simulink model "Hopper_3DOF_v1_9_J"  (R2025a)
settings: Solver=VariableStepAuto  StartTime=0.0  StopTime=20  RelTol=1e-3
values from neighbouring files (symbols this model uses):
  g = 9.80665    [vehicle_info.m]
  I = [ I_xx, 0,     0 ... (first row only)    [vehicle_info.m]
  m0 = 48    [vehicle_info.m]
  mdot = 0    [vehicle_info.m]
  mt = 114    [vehicle_info.m]
undefined symbols (not defined in the file or in its folder): bp, tbl
libraries: aerolibanim x3, aerolibobsolete x1, simulink_extras x1, slpidlib x1, simulink x1, SignalEditorBlockLib x1
settings Model: Creator=vip  LastModifiedBy=asing
settings SolverCC: ZeroCrossAlgorithm=Adaptive
settings DebuggingCC: IgnoredZcDiagnostic=none

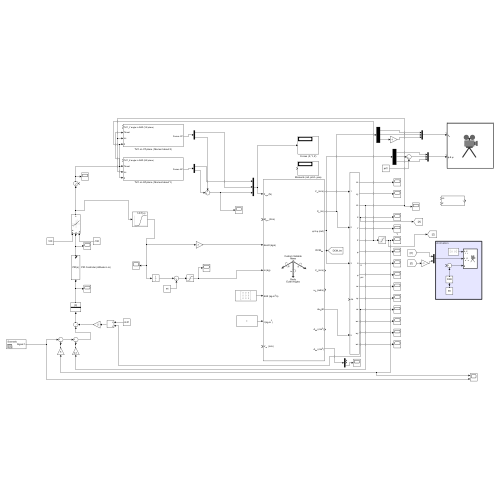
[thumbnail: Simulink's stored preview of the top-level diagram]
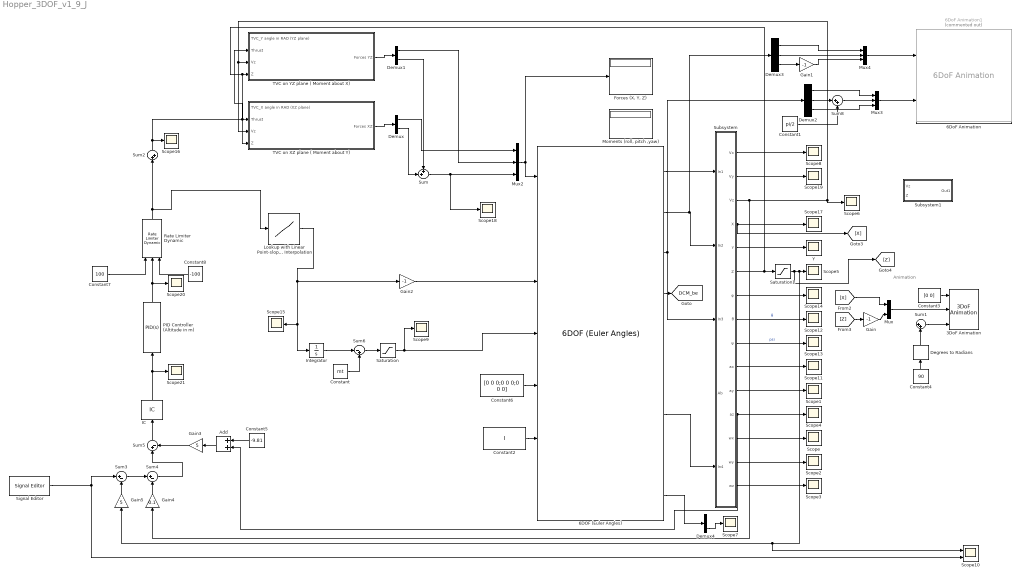
== system Hopper_3DOF_v1_9_J ==
  note: Animation
  3DoF Animation : aerolibanim/3DoF Animation  u1=[-5 5 -10 10 -250 0]  u2=0.05  u3=0.1  u5=Fly alongside  u6=[10 10 0]  u7=70  u8=off
  6DOF (Euler Angles) : aerolibobsolete/6DOF (Euler Angles)  units=Metric (MKS)  mtype=Custom Variable  rep=Euler Angles  xme_0=[0 0 0]  Vm_0=[0 0 0]  eul_0=[0 0 0]  pm_0=[0 0 0]  mass_0=4  mass_e=0.5  mass_f=2.0  inertia=[43 0 0 ; 0 43 0; 0 0 43]  inertia_e=eye(3)  inertia_f=2*eye(3)  k_quat=1.0  vre_flag=on  abi_flag=on  aMode=0  xme_statename=''  Vm_statename=''  eul_statename=''  quat_statename=''  pm_statename=''  mass_statename=''
  6DoF Animation : aerolibanim/6DoF Animation  u1=[-5 5 -10 10 -250 0]  u2=0.05  u3=5  u4=[40 0 -50]  u5=Fly alongside  u6=[10 10 0]  u7=70  u8=on
  6DoF Animation1 : aerolibanim/6DoF Animation  Commented=on  u1=[-5 5 -10 10 -250 0]  u2=0.05  u3=5  u4=[40 0 -50]  u5=Fly alongside  u6=[10 10 0]  u7=70  u8=on
  Add : Sum
  Constant : Constant  Value=mt
  Constant1 : Constant  Value=pi/2
  Constant2 : Constant  Value=I
  Constant3 : Constant  Value=[0 0]
  Constant4 : Constant  Value=90
  Constant5 : Constant  Value=-9.81
  Constant6 : Constant  Value=[0 0 0;0 0 0;0 0 0]
  Constant7 : Constant  Value=100  SampleTime=-1
  Constant8 : Constant  Value=-100  SampleTime=-1
  Degrees to Radians : simulink_extras/Transformations/Degrees to Radians
  Demux : Demux  Outputs=2
  Demux1 : Demux  Outputs=2
  Demux2 : Demux  Outputs=3
  Demux3 : Demux  Outputs=3
  Demux4 : Demux  Outputs=3
  "Forces (X, Y, Z)" : Display
  Gain : Gain  Gain=-1
  Gain1 : Gain  Gain=-1
  Gain2 : Gain  Gain=-1
  Gain3 : Gain  Gain=5
  Gain4 : Gain  Gain=0.1
  Gain5 : Gain  Gain=5
  IC : InitialCondition  Value=0
  Integrator : Integrator
  Lookup with Linear Point-slope Interpolation : Lookup_n-D  NumberOfTableDimensions=1  BreakpointsForDimension1=bp  Table=tbl  InternalRulePriority=Speed  RndMeth=Simplest
  "Moments (roll, pitch ,yaw)" : Display
  Mux : Mux  Inputs=2
  Mux2 : Mux  Inputs=3
  Mux3 : Mux  Inputs=3
  Mux4 : Mux  Inputs=3
  PID Controller (Altitude in m) : slpidlib/PID Controller  Controller=PID  Form=Parallel  TimeDomain=Continuous-time  UseExternalTs=off  SampleTime=-1  IntegratorMethod=Forward Euler  FilterMethod=Forward Euler  ControllerParametersSource=internal  P=10  I=0.8  UseKiTs=off  D=50  UseExternalDerivativeSource=off  N=50  UseFilter=on  TunerSelectOption=Transfer Function Based (PID Tuner App)  InitialConditionSource=internal  InitialConditionForIntegrator=890  InitialConditionForFilter=890  DifferentiatorICPrevScaledInput=0  ExternalReset=none  TrackingMode=off  Kt=1  LimitOutput=on  SatLimitsSource=internal  UpperSaturationLimit=2400  LowerSaturationLimit=890  LinearizeAsGain=off  AntiWindupMode=clamping  Kb=1  LimitIntegrator=on  UpperIntegratorSaturationLimit=2400  LowerIntegratorSaturationLimit=890  POutMin=[]  POutMax=[]  IOutMin=[]  IOutMax=[]  DOutMin=[]  DOutMax=[]  NOutMin=[]  NOutMax=[]  SumOutMin=[]  SumOutMax=[]  SaturationOutMin=[]  SaturationOutMax=[]  PParamMin=[]  PParamMax=[]  IParamMin=[]  IParamMax=[]  DParamMin=[]  DParamMax=[]  NParamMin=[]  NParamMax=[]  KbParamMin=[]  KbParamMax=[]  KtParamMin=[]  KtParamMax=[]  KbOutMin=[]  KbOutMax=[]  KtOutMin=[]  KtOutMax=[]  IntegratorOutMin=[]  IntegratorOutMax=[]  FilterOutMin=[]  FilterOutMax=[]  SumI1OutMin=[]  SumI1OutMax=[]  SumI2OutMin=[]  SumI2OutMax=[]  SumI3OutMin=[]  SumI3OutMax=[]  SumI4OutMin=[]  SumI4OutMax=[]  SumDOutMin=[]  SumDOutMax=[]  DifferentiatorOutMin=[]  DifferentiatorOutMax=[]  FilterDiffOutCoefMin=[]  FilterDiffOutCoefMax=[]  ReciprocalOutMin=[]  ReciprocalOutMax=[]  SumDenOutMin=[]  SumDenOutMax=[]  SumNumOutMin=[]  SumNumOutMax=[]  DivideOutMin=[]  DivideOutMax=[]  UdiffTsProdOutMin=[]  UdiffTsProdOutMax=[]  NTsProdOutMin=[]  NTsProdOutMax=[]  UintegralTsProdOutMin=[]  UintegralTsProdOutMax=[]  UngainTsProdOutMin=[]  UngainTsProdOutMax=[]  ClampingZeroOutDataTypeStr=Inherit: Inherit via back propagation  ClampingZeroOutMin=[]  ClampingZeroOutMax=[]  FilterDenConstantOutDataTypeStr=Inherit: Inherit via back propagation  FilterDenConstantOutMin=[]  FilterDenConstantOutMax=[]  PCopyOutDataTypeStr=Inherit: Inherit via back propagation  PCopyOutMin=[]  PCopyOutMax=[]  NCopyOutDataTypeStr=Inherit: Inherit via back propagation  NCopyOutMin=[]  NCopyOutMax=[]  IntegratorContinuousStateAttributes=''  IntegratorStateMustResolveToSignalObject=off  IntegratorRTWStateStorageClass=Auto  FilterContinuousStateAttributes=''  FilterStateMustResolveToSignalObject=off  FilterRTWStateStorageClass=Auto  ParallelPVariant=InternalParameters  IdealPVariant=Disabled  IVariant=InternalParameters  DVariant=InternalParameters  IntegratorVariant=Continuous  SatVariant=Enabled  AWVariant=ContClampingParallel  PCopyVariant=Disabled  TRVariant=Disabled  FdbkBlocksVariant=Forward  IdealPFdbkVariant=Disabled  SatFdbkVariant=Disabled  DerivativeFilterVariant=ContFilter  NVariant=InternalParameters  NCopyVariant=Disabled  FilterICVariant=InternalICsFilter  IntegratorICVariant=InternalICs  ExternalResetVariant=Disabled  TRSumVariant=Passthrough  SumFdbkVariant=Disabled  SumVariant=Sum_PID  TsampFilterVariant=InternalTs  TsampNgainVariant=Passthrough  TsampIntegralVariant=Disabled_SignalSpec  ExternalSaturationOutDataTypeStr=Inherit: Same as second input  DerivativeSourceVariant=ErrorSignal  PreIntVariant=InternalPreInt
  Rate Limiter Dynamic : simulink/Discontinuities/Rate Limiter Dynamic
  Saturation : Saturate  UpperLimit=mt  LowerLimit=m0
  Saturation1 : Saturate  UpperLimit=inf  LowerLimit=0
  Scope{,1..9,11..21} (21 alike) : Scope
      Scope settings: ActiveDisplayYMinimum=-1  ActiveDisplayYMaximum=1  DataLoggingVariableName=ScopeData10
      Scope1 settings: ActiveDisplayYMinimum=-1  ActiveDisplayYMaximum=1
      Scope11 settings: ActiveDisplayYMinimum=-1  ActiveDisplayYMaximum=1  DataLoggingVariableName=ScopeData6
      Scope12 settings: ActiveDisplayYMinimum=-0.01376  ActiveDisplayYMaximum=0.12381  DataLoggingVariableName=ScopeData7
      Scope13 settings: ActiveDisplayYMinimum=-1  ActiveDisplayYMaximum=1  DataLoggingVariableName=ScopeData8
      Scope14 settings: ActiveDisplayYMinimum=-0.40362  ActiveDisplayYMaximum=0.917  DataLoggingVariableName=ScopeData9
      Scope15 settings: ActiveDisplayYMinimum=0.4060620759659761  ActiveDisplayYMaximum=0.71681974522320513  DataLoggingVariableName=ScopeData15
      Scope16 settings: ActiveDisplayYMinimum=-1  ActiveDisplayYMaximum=1  DataLoggingVariableName=ScopeData17
      Scope17 settings: ActiveDisplayYMinimum=-0.03461  ActiveDisplayYMaximum=0.31153  DataLoggingVariableName=ScopeData4
      Scope18 settings: ActiveDisplayYMinimum=-393.49560759392443  ActiveDisplayYMaximum=1261.879468345322  DataLoggingVariableName=ScopeData18
      Scope19 settings: ActiveDisplayYMinimum=-1  ActiveDisplayYMaximum=1  DataLoggingVariableName=ScopeData16
      Scope2 settings: ActiveDisplayYMinimum=-0.01484  ActiveDisplayYMaximum=0.12541  DataLoggingVariableName=ScopeData11
      Scope20 settings: ActiveDisplayYMinimum=876.2815931984652  ActiveDisplayYMaximum=1068.8739039399095  DataLoggingVariableName=ScopeData22
      Scope21 settings: ActiveDisplayYMinimum=-55.4130507317401  ActiveDisplayYMaximum=57.561717444849705  DataLoggingVariableName=ScopeData23
      Scope3 settings: ActiveDisplayYMinimum=-1  ActiveDisplayYMaximum=1  DataLoggingVariableName=ScopeData12
      Scope4 settings: ActiveDisplayYMinimum=-0.67950402962173528  ActiveDisplayYMaximum=0.67417469443563827  DataLoggingVariableName=ScopeData5
      Scope5 settings: ActiveDisplayYMinimum=-5.4800664649435831  ActiveDisplayYMaximum=49.320598184492255
      Scope6 settings: ActiveDisplayYMinimum=-2.3884313283725929  ActiveDisplayYMaximum=3.709340437820893  DataLoggingVariableName=ScopeData2
      Scope7 settings: ActiveDisplayYMinimum=-2.6790448009064565  ActiveDisplayYMaximum=4.1150786467546157  DataLoggingVariableName=ScopeData13
      Scope8 settings: ActiveDisplayYMinimum=-1  ActiveDisplayYMaximum=1  DataLoggingVariableName=ScopeData4
      Scope9 settings: ActiveDisplayYMinimum=39.75  ActiveDisplayYMaximum=122.25  DataLoggingVariableName=ScopeData14
  Scope10 : Scope  NumInputPorts=2
      settings: ActiveDisplayYMinimum=-5.2268980176886384  ActiveDisplayYMaximum=42.5440387764437  DataLoggingVariableName=ScopeData3
  Signal Editor : SignalEditorBlockLib/Signal Editor  FileName=trajectory_1.mat  ActiveScenario=Scenario  ActiveSignal=Signal 1  IsBus=off  OutputBusObjectStr=Bus: BusObject  SampleTime=0  ZeroCross=off  OutputAfterFinalValue=Setting to zero  Unit=inherit  PreserveSignalName=on  ApplySigPropsToAllScenarios=on  ApplySigPropsToAllSignals=off  SignalPropertySource=Dialog parameters
  Subsystem : Subsystem
  Subsystem1 : Subsystem
  Sum : Sum  Inputs=++|
  Sum1 : Sum  Inputs=|++
  Sum2 : Sum  Inputs=|++
  Sum3 : Sum  Inputs=|+-
  Sum4 : Sum  Inputs=|+-
  Sum5 : Sum  Inputs=|+-
  Sum6 : Sum  Inputs=|-+
  Sum8 : Sum  Inputs=|++
  TVC on XZ plane ( Moment about Y) : Subsystem
  TVC on YZ plane ( Moment about X) : Subsystem
  Y : Scope
      settings: ActiveDisplayYMinimum=-0.22309  ActiveDisplayYMaximum=1.9929  DataLoggingVariableName=ScopeData20
  tag scope: DCM_be=global
  wires:
  Constant6/1 -> 6DOF (Euler Angles)/5
  6DOF (Euler Angles)/4 -> [DCM_be]
  Constant3/1 -> 3DoF Animation/1
  Mux/1 -> 3DoF Animation/2
  Subsystem/4(X) -> Scope17/1, [X]
  6DOF (Euler Angles)/1 -> Subsystem/1(In1)
  6DOF (Euler Angles)/3 -> Demux2/1, Subsystem/3(In3)
  6DOF (Euler Angles)/7 -> Subsystem/5(In4)
  Subsystem/1(Vx) -> Scope8/1
  Subsystem/2(Vy) -> Scope19/1
  Subsystem/5(Y) -> Y/1
  Subsystem/7(φ) -> Scope14/1
  Subsystem/10(ax) -> Scope11/1
  Subsystem/11(ay) -> Scope1/1
  Subsystem/12(az) -> Add/2, Scope4/1
  Subsystem/13(wx) -> Scope/1
  Subsystem/14(wy) -> Scope2/1
  Subsystem/15(wz) -> Scope3/1
  [X] -> Mux/1
  [Z] -> Gain/1
  Mux2/1 -> "Forces (X, Y, Z)"/1, 6DOF (Euler Angles)/1
  Gain/1 -> Mux/2
  Constant4/1 -> Degrees to Radians/1
  Degrees to Radians/1 -> Sum1/2
  Sum1/1 -> 3DoF Animation/3
  Signal Editor/1 -> Sum3/1, Scope10/2
  Subsystem/9(ψ) -> Scope13/1  "psi"
  Sum6/1 -> Saturation/1
  Lookup with Linear Point-slope Interpolation/1 -> Scope15/1, Integrator/1, Gain2/1
  Constant/1 -> Sum6/2
  Saturation/1 -> Scope9/1, 6DOF (Euler Angles)/4
  Demux2/2 -> Sum8/1
  Constant1/1 -> Sum8/2
  Mux3/1 -> 6DoF Animation/2
  Demux2/1 -> Mux3/1
  Sum8/1 -> Mux3/2
  Demux2/3 -> Mux3/3
  Demux3/2 -> Mux4/2
  6DOF (Euler Angles)/2 -> Demux3/1, Subsystem/2(In2)
  Demux3/3 -> Gain1/1
  Mux4/1 -> 6DoF Animation/1
  Demux3/1 -> Mux4/1
  Gain1/1 -> Mux4/3
  Subsystem/8(θ) -> Scope12/1  "θ"
  Demux1/1 -> Mux2/2
  TVC on XZ plane ( Moment about Y)/1(Forces XZ) -> Demux/1
  Demux/2 -> Sum/2
  Demux1/2 -> Sum/1
  Demux/1 -> Mux2/1
  TVC on YZ plane ( Moment about X)/1(Forces YZ) -> Demux1/1
  Constant2/1 -> 6DOF (Euler Angles)/6
  6DOF (Euler Angles)/9 -> Demux4/1
  Demux4/3 -> Scope7/1
  Gain2/1 -> 6DOF (Euler Angles)/3
  Rate Limiter Dynamic/1 -> Sum2/1, Lookup with Linear Point-slope Interpolation/1
  IC/1 -> Scope21/1, PID Controller (Altitude in m)/1
  Constant7/1 -> Rate Limiter Dynamic/1
  Constant8/1 -> Rate Limiter Dynamic/3
  Sum/1 -> Scope18/1, Mux2/3
  Subsystem/3(Vz) -> Gain4/1, Scope6/1, TVC on XZ plane ( Moment about Y)/3(Vz), TVC on YZ plane ( Moment about X)/3(Vz)
  Subsystem/6(Z) -> TVC on XZ plane ( Moment about Y)/4(Z), TVC on YZ plane ( Moment about X)/4(Z), Saturation1/1
  Saturation1/1 -> Scope5/1, Scope10/1, Gain5/1, [Z]
  Integrator/1 -> Sum6/1
  Sum2/1 -> Scope16/1, TVC on YZ plane ( Moment about X)/2(Thrust), TVC on XZ plane ( Moment about Y)/2(Thrust)
  Sum3/1 -> Sum4/1
  Sum4/1 -> Sum5/1
  Sum5/1 -> IC/1
  Gain3/1 -> Sum5/2
  Gain4/1 -> Sum4/2
  Gain5/1 -> Sum3/2
  Constant5/1 -> Add/1
  Add/1 -> Gain3/1
  PID Controller (Altitude in m)/1 -> Scope20/1, Rate Limiter Dynamic/2

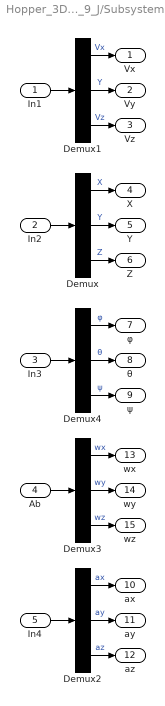
== system Hopper_3DOF_v1_9_J/Subsystem ==
  In1 : Inport
  In2 : Inport  Port=2
  In3 : Inport  Port=3
  Ab : Inport  Port=4
  In4 : Inport  Port=5
  Demux{,1..4} (5 alike) : Demux  Outputs=3
  Vx : Outport
  Vy : Outport  Port=2
  Vz : Outport  Port=3
  X : Outport  Port=4
  Y : Outport  Port=5
  Z : Outport  Port=6
  φ : Outport  Port=7
  θ : Outport  Port=8
  ψ : Outport  Port=9
  ax : Outport  Port=10
  ay : Outport  Port=11
  az : Outport  Port=12
  wx : Outport  Port=13
  wy : Outport  Port=14
  wz : Outport  Port=15
  wires:
  Demux/3 -> Z/1  "Z"
  Demux4/1 -> φ/1  "φ"
  In2/1 -> Demux/1
  In4/1 -> Demux2/1
  Demux/2 -> Y/1  "Y"
  Demux/1 -> X/1  "X"
  Demux1/3 -> Vz/1  "Vz"
  Demux1/1 -> Vx/1  "Vx"
  Demux4/3 -> ψ/1  "ψ"
  Demux4/2 -> θ/1  "θ"
  Demux2/2 -> ay/1  "ay"
  In1/1 -> Demux1/1
  In3/1 -> Demux4/1
  Demux2/3 -> az/1  "az"
  Demux2/1 -> ax/1  "ax"
  Demux1/2 -> Vy/1  "Y"
  Demux3/1 -> wx/1  "wx"
  Demux3/3 -> wz/1  "wz"
  Demux3/2 -> wy/1  "wy"
  Ab/1 -> Demux3/1

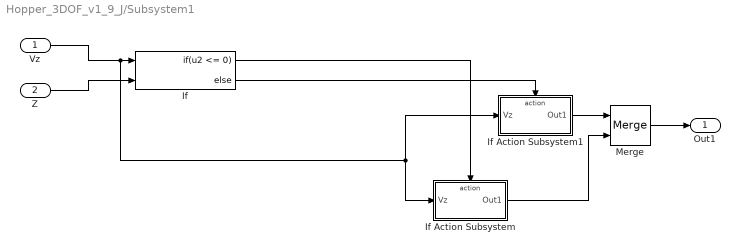
== system Hopper_3DOF_v1_9_J/Subsystem1 ==
  Vz : Inport
  Z : Inport  Port=2
  If : If  NumInputs=2  IfExpression=u2 <= 0
  If Action Subsystem : Subsystem  TreatAsAtomicUnit=on
  If Action Subsystem1 : Subsystem  TreatAsAtomicUnit=on
  Merge : Merge
  Out1 : Outport
  wires:
  Vz/1 -> If Action Subsystem1/1(Vz), If Action Subsystem/1(Vz), If/1
  Z/1 -> If/2
  If/1 -> If Action Subsystem/Action
  If/2 -> If Action Subsystem1/Action
  If Action Subsystem/1(Out1) -> Merge/2
  If Action Subsystem1/1(Out1) -> Merge/1
  Merge/1 -> Out1/1

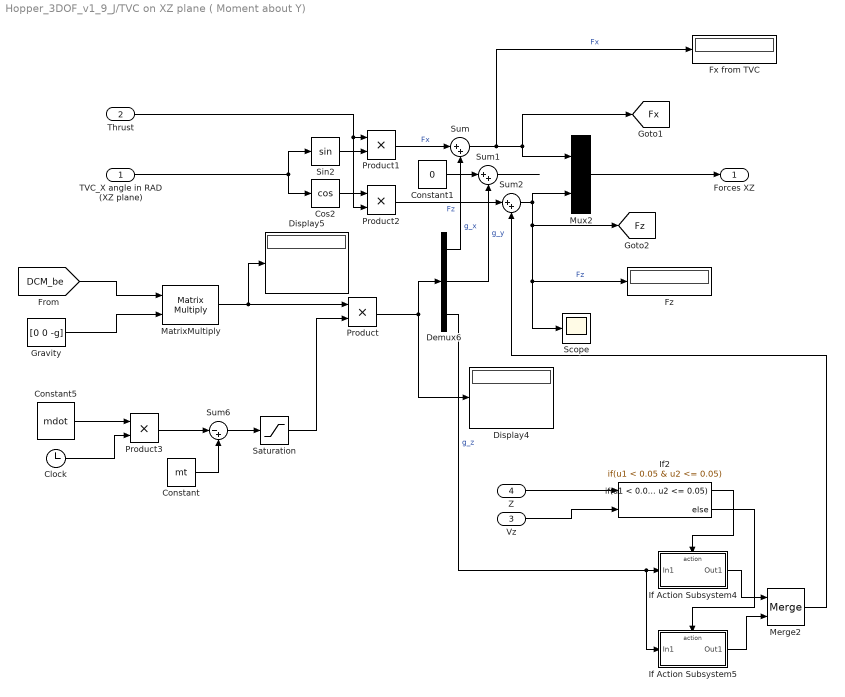
== system Hopper_3DOF_v1_9_J/TVC on XZ plane ( Moment about Y) ==
  TVC_X angle in RAD (XZ plane) : Inport
  Thrust : Inport  Port=2
  Vz : Inport  Port=3
  Z : Inport  Port=4
  Clock : Clock
  Constant : Constant  Value=mt
  Constant1 : Constant  Value=0
  Constant5 : Constant  Value=mdot
  Cos2 : Trigonometry  Operator=cos
  Demux6 : Demux  Outputs=3
  Display4 : Display
  Display5 : Display
  "Fx from TVC " : Display
  "Fz " : Display
  Gravity : Constant  Value=[0 0 -g]
  If Action Subsystem4 : Subsystem  TreatAsAtomicUnit=on
  If Action Subsystem5 : Subsystem  TreatAsAtomicUnit=on
  If2 : If  NumInputs=2  IfExpression=u1 < 0.05 & u2 <= 0.05  ZeroCross=off
  MatrixMultiply : Product  Multiplication=Matrix(*)
  Merge2 : Merge
  Mux2 : Mux  Inputs=2
  Product{,1..3} (4 alike) : Product
  Saturation : Saturate  UpperLimit=mt  LowerLimit=m0
  Scope : Scope
      settings: ActiveDisplayYMinimum=-352.54531543215779  ActiveDisplayYMaximum=919.02113985366293  DataLoggingVariableName=ScopeData21
  Sin2 : Trigonometry
  Sum : Sum  Inputs=|++
  Sum1 : Sum  Inputs=|++
  Sum2 : Sum  Inputs=|++
  Sum6 : Sum  Inputs=|-+
  Forces XZ : Outport
  tag scope: Fx=global, Fz=global
  wires:
  Product/1 -> Demux6/1, Display4/1
  Mux2/1 -> Forces XZ/1
  TVC_X angle in RAD (XZ plane)/1 -> Cos2/1, Sin2/1
  Product1/1 -> Sum/1  "Fx"
  Sum1/1 -> ?
  Sin2/1 -> Product1/2
  Thrust/1 -> Product2/2, Product1/1
  MatrixMultiply/1 -> Display5/1, Product/1
  Sum/1 -> "Fx from TVC "/1, [Fx], Mux2/1  "Fx"
  Product2/1 -> Sum2/1  "Fz"
  Sum2/1 -> Scope/1, "Fz "/1, [Fz], Mux2/2  "Fz"
  Constant1/1 -> Sum1/1
  [DCM_be] -> MatrixMultiply/1
  Gravity/1 -> MatrixMultiply/2
  Demux6/2 -> Sum1/2  "g_y"
  Demux6/1 -> Sum/2  "g_x"
  Cos2/1 -> Product2/1
  Saturation/1 -> Product/2
  Product3/1 -> Sum6/1
  Constant5/1 -> Product3/1
  Sum6/1 -> Saturation/1
  Constant/1 -> Sum6/2
  Clock/1 -> Product3/2
  If2/1 -> If Action Subsystem4/Action
  If Action Subsystem5/1(Out1) -> Merge2/2
  Vz/1 -> If2/2
  If2/2 -> If Action Subsystem5/Action
  Z/1 -> If2/1
  If Action Subsystem4/1(Out1) -> Merge2/1
  Demux6/3 -> If Action Subsystem5/1(In1), If Action Subsystem4/1(In1)  "g_z"
  Merge2/1 -> Sum2/2

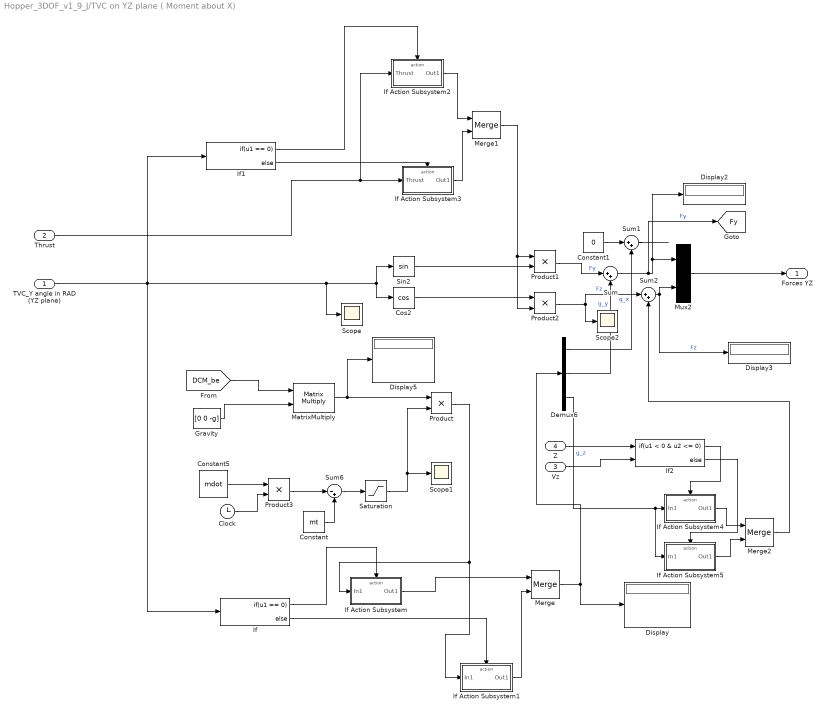
== system Hopper_3DOF_v1_9_J/TVC on YZ plane ( Moment about X) ==
  TVC_Y angle in RAD (YZ plane) : Inport
  Thrust : Inport  Port=2
  Vz : Inport  Port=3
  Z : Inport  Port=4
  Clock : Clock
  Constant : Constant  Value=mt
  Constant1 : Constant  Value=0
  Constant5 : Constant  Value=mdot
  Cos2 : Trigonometry  Operator=cos
  Demux6 : Demux  Outputs=3
  Display{,2..3,5} (4 alike) : Display
  Gravity : Constant  Value=[0 0 -g]
  If : If  IfExpression=u1 == 0
  If Action Subsystem : Subsystem  TreatAsAtomicUnit=on
  If Action Subsystem1 : Subsystem  TreatAsAtomicUnit=on
  If Action Subsystem2 : Subsystem  TreatAsAtomicUnit=on
  If Action Subsystem3 : Subsystem  TreatAsAtomicUnit=on
  If Action Subsystem4 : Subsystem  TreatAsAtomicUnit=on
  If Action Subsystem5 : Subsystem  TreatAsAtomicUnit=on
  If1 : If  IfExpression=u1 == 0
  If2 : If  NumInputs=2  IfExpression=u1 < 0 & u2 <= 0  ZeroCross=off
  MatrixMultiply : Product  Multiplication=Matrix(*)
  Merge : Merge
  Merge1 : Merge
  Merge2 : Merge
  Mux2 : Mux  Inputs=2
  Product{,1..3} (4 alike) : Product
  Saturation : Saturate  UpperLimit=mt  LowerLimit=m0
  Scope : Scope
      settings: ActiveDisplayYMinimum=-1  ActiveDisplayYMaximum=1  DataLoggingVariableName=ScopeData3
  Scope1 : Scope
      settings: ActiveDisplayYMinimum=45  ActiveDisplayYMaximum=75
  Scope2 : Scope
      settings: ActiveDisplayYMinimum=-1  ActiveDisplayYMaximum=1  DataLoggingVariableName=ScopeData19
  Sin2 : Trigonometry
  Sum : Sum  Inputs=|++
  Sum1 : Sum  Inputs=|++
  Sum2 : Sum  Inputs=|++
  Sum6 : Sum  Inputs=|-+
  Forces YZ : Outport
  tag scope: Fy=global
  wires:
  Cos2/1 -> Product2/1
  Demux6/1 -> Sum1/2  "g_x"
  Demux6/2 -> Sum/2  "g_y"
  Constant1/1 -> Sum1/1
  Sum2/1 -> Mux2/2, Display3/1  "Fz"
  Product2/1 -> Scope2/1, Sum2/1  "Fz"
  Sum/1 -> [Fy], Mux2/1, Display2/1  "Fy"
  Sin2/1 -> Product1/2
  Sum1/1 -> ?
  Product1/1 -> Sum/1  "Fy"
  TVC_Y angle in RAD (YZ plane)/1 -> If1/1, Scope/1, Sin2/1, Cos2/1, If/1
  Mux2/1 -> Forces YZ/1
  Product/1 -> If Action Subsystem1/1(In1), If Action Subsystem/1(In1)
  MatrixMultiply/1 -> Product/1, Display5/1
  [DCM_be] -> MatrixMultiply/1
  Sum6/1 -> Saturation/1
  Constant/1 -> Sum6/2
  Gravity/1 -> MatrixMultiply/2
  Product3/1 -> Sum6/1
  Saturation/1 -> Product/2, Scope1/1
  Constant5/1 -> Product3/1
  Clock/1 -> Product3/2
  If/1 -> If Action Subsystem/Action
  If Action Subsystem/1(Out1) -> Merge/1
  If Action Subsystem1/1(Out1) -> Merge/2
  If/2 -> If Action Subsystem1/Action
  Merge/1 -> Demux6/1, Display/1
  Thrust/1 -> If Action Subsystem2/1(Thrust), If Action Subsystem3/1(Thrust)
  If Action Subsystem2/1(Out1) -> Merge1/1
  If1/1 -> If Action Subsystem2/Action
  If Action Subsystem3/1(Out1) -> Merge1/2
  If1/2 -> If Action Subsystem3/Action
  Merge1/1 -> Product1/1, Product2/2
  Z/1 -> If2/1
  Vz/1 -> If2/2
  If2/1 -> If Action Subsystem4/Action
  Demux6/3 -> If Action Subsystem5/1(In1), If Action Subsystem4/1(In1)  "g_z"
  If2/2 -> If Action Subsystem5/Action
  If Action Subsystem4/1(Out1) -> Merge2/1
  If Action Subsystem5/1(Out1) -> Merge2/2
  Merge2/1 -> Sum2/2

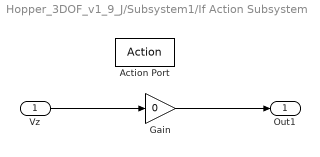
== system Hopper_3DOF_v1_9_J/Subsystem1/If Action Subsystem ==
  Vz : Inport
  Action Port : ActionPort  ActionPortLabel=if(u2 <= 0)
  Gain : Gain  Gain=0
  Out1 : Outport
  wires:
  Vz/1 -> Gain/1
  Gain/1 -> Out1/1

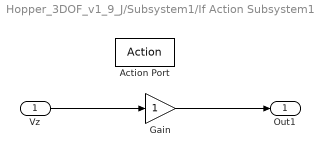
== system Hopper_3DOF_v1_9_J/Subsystem1/If Action Subsystem1 ==
  Vz : Inport
  Action Port : ActionPort  ActionPortLabel=else
  Gain : Gain
  Out1 : Outport
  wires:
  Vz/1 -> Gain/1
  Gain/1 -> Out1/1

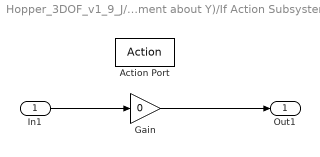
== system Hopper_3DOF_v1_9_J/TVC on XZ plane ( Moment about Y)/If Action Subsystem4 ==
  In1 : Inport
  Action Port : ActionPort  ActionPortLabel=if(u1 < 0.05 & u2 <= 0.05)
  Gain : Gain  Gain=0
  Out1 : Outport
  wires:
  In1/1 -> Gain/1
  Gain/1 -> Out1/1

== system Hopper_3DOF_v1_9_J/TVC on XZ plane ( Moment about Y)/If Action Subsystem5 ==
  In1 : Inport
  Action Port : ActionPort  ActionPortLabel=else
  Out1 : Outport
  wires:
  In1/1 -> Out1/1

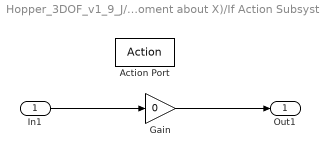
== system Hopper_3DOF_v1_9_J/TVC on YZ plane ( Moment about X)/If Action Subsystem ==
  In1 : Inport
  Action Port : ActionPort  ActionPortLabel=if(u1 == 0)
  Gain : Gain  Gain=0
  Out1 : Outport
  wires:
  In1/1 -> Gain/1
  Gain/1 -> Out1/1

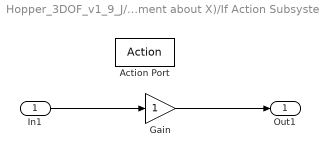
== system Hopper_3DOF_v1_9_J/TVC on YZ plane ( Moment about X)/If Action Subsystem1 ==
  In1 : Inport
  Action Port : ActionPort  ActionPortLabel=else
  Gain : Gain
  Out1 : Outport
  wires:
  Gain/1 -> Out1/1
  In1/1 -> Gain/1

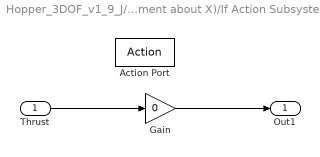
== system Hopper_3DOF_v1_9_J/TVC on YZ plane ( Moment about X)/If Action Subsystem2 ==
  Thrust : Inport
  Action Port : ActionPort  ActionPortLabel=if(u1 == 0)
  Gain : Gain  Gain=0
  Out1 : Outport
  wires:
  Thrust/1 -> Gain/1
  Gain/1 -> Out1/1

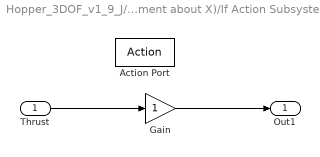
== system Hopper_3DOF_v1_9_J/TVC on YZ plane ( Moment about X)/If Action Subsystem3 ==
  Thrust : Inport
  Action Port : ActionPort  ActionPortLabel=else
  Gain : Gain
  Out1 : Outport
  wires:
  Gain/1 -> Out1/1
  Thrust/1 -> Gain/1

== system Hopper_3DOF_v1_9_J/TVC on YZ plane ( Moment about X)/If Action Subsystem4 ==
  In1 : Inport
  Action Port : ActionPort  ActionPortLabel=if(u1 < 0 & u2 <= 0)
  Gain : Gain  Gain=0
  Out1 : Outport
  wires:
  In1/1 -> Gain/1
  Gain/1 -> Out1/1

== system Hopper_3DOF_v1_9_J/TVC on YZ plane ( Moment about X)/If Action Subsystem5 ==
  In1 : Inport
  Action Port : ActionPort  ActionPortLabel=else
  Out1 : Outport
  wires:
  In1/1 -> Out1/1
